simulink model "A_ZH_Z5"  (R2026a)
settings: Solver=ode45  StopTime=10e-3  MaxStep=25e-6/25  EnableMultiTasking=on
settings Model: Creator=oktato  LastModifiedBy=Szalay
settings HardwareCC: ProdHWDeviceType=32-bit Generic

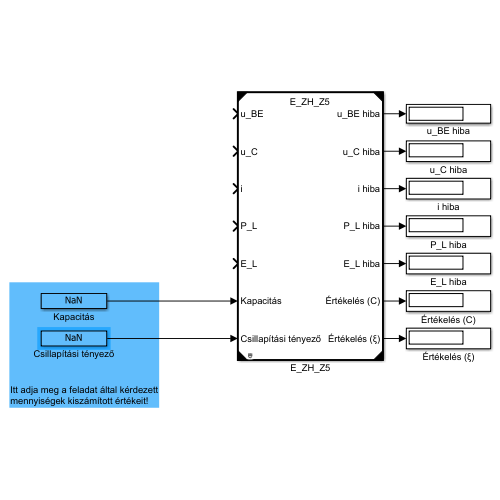
[thumbnail: Simulink's stored preview of the top-level diagram]
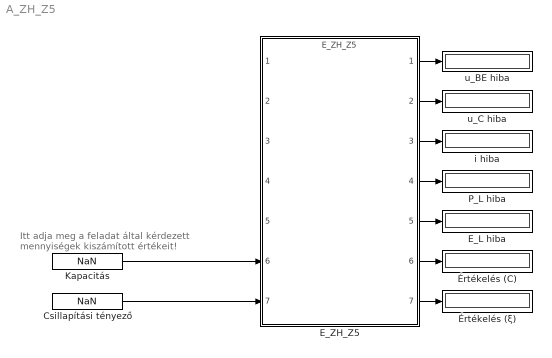
== system A_ZH_Z5 ==
  note: Itt adja meg a feladat által kérdezett
      | mennyiségek kiszámított értékeit!
  Csillapítási tényező : Constant  Value=NaN
  E_L hiba : Display
  E_ZH_Z5 : ModelReference  ModelNameDialog=E_ZH_Z5.slxp  ModelReferenceVersion=3.7  CopyOfModelProtected=on
  Kapacitás : Constant  Value=NaN
  P_L hiba : Display
  i hiba : Display
  u_BE hiba : Display
  u_C hiba : Display
  Értékelés (C) : Display
  Értékelés (ξ) : Display
  wires:
  E_ZH_Z5/3 -> i hiba/1
  E_ZH_Z5/1 -> u_BE hiba/1
  E_ZH_Z5/2 -> u_C hiba/1
  Kapacitás/1 -> E_ZH_Z5/6
  Csillapítási tényező/1 -> E_ZH_Z5/7
  E_ZH_Z5/7 -> Értékelés (ξ)/1
  E_ZH_Z5/6 -> Értékelés (C)/1
  E_ZH_Z5/4 -> P_L hiba/1
  E_ZH_Z5/5 -> E_L hiba/1
